simulink model "turbo_controller"  (R2025a)
settings: Solver=FixedStepAuto  StartTime=0.0  StopTime=inf  FixedStep=0.001  RelTol=1e-3
PostLoadFcn:
  | % 自动定位同目录CubeMX文件；不需要外部初始化脚本。
  | codertarget.data.setParameterValue('turbo_controller','STM32CubeMX.ProjectFile',fullfile(fileparts(get_param('turbo_controller','FileName')),'turbo_f407.ioc'));
InitFcn:
  | % 中文说明：按原控制器字段与类型创建三组接口总线；控制参数已内嵌。
  | tc_names=["EValve_Cycle" "EValve_Open" "Eblast_Cycle" "Eblast_Open" "Motor_Cycle" "Motor_Open" "EValve_Enable" "Eblast_Enable" "Motor_Enable" "SWO_Firework" "SWO_BleedAir" "EngineState" "Flag_ECUReset_Clear" "Flag_ECUReset_Save" "Flag_Reset_Enable" "Accelerator" "Nc_dem" "Nc"]; tc_types=["uint16" "uint16" "uint16" "uint16" "uint16" "uint16" "uint8" "uint8" "uint8" "uint8" "uint8" "uint8" "uint8" "uint8" "uint8" "single" "single" "single"];
  | for tc_k=1:numel(tc_names)
  |  tc_e(tc_k)=Simulink.BusElement; tc_e(tc_k).Name=char(tc_names(tc_k)); tc_e(tc_k).DataType=char(tc_types(tc_k));
  | end
  | EngineControl_Out=Simulink.Bus; EngineControl_Out.DataScope='Exported'; EngineControl_Out.Elements=tc_e;
  | clear tc_e tc_names tc_types tc_k
  | tc_names=["savedata1" "savedata2" "savedata3" "savedata4" "savedata5" "savedata6" "savedata7" "savedata8" "savedata9" "savedata10" "savedata11" "savedata12" "savedata13" "savedata14" "savedata15" "savedata16" "savedata17" "savedata18" "savedata19" "savedata20" "savedata21" "savedata22" "savedata23" "savedata24" "savedata25"]; tc_types=["single" "single" "single" "single" "single" "single" "single" "single" "single" "single" "single" "single" "single" "single" "single" "single" "single" "single" "single" "single" "single" "single" "single" "single" "single"];
  | for tc_k=1:numel(tc_names)
  |  tc_e(tc_k)=Simulink.BusElement; tc_e(tc_k).Name=char(tc_names(tc_k)); tc_e(tc_k).DataType=char(tc_types(tc_k));
  | end
  | SaveData_Out=Simulink.Bus; SaveData_Out.DataScope='Exported'; SaveData_Out.Elements=tc_e;
  | clear tc_e tc_names tc_types tc_k
  | tc_names=["senddata1" "senddata2" "senddata3" "senddata4" "senddata5" "senddata6" "senddata7" "senddata8" "senddata9" "senddata10" "senddata11" "senddata12" "senddata13" "senddata14" "senddata15" "senddata16" "senddata17" "senddata18" "senddata19" "senddata20" "senddata21" "senddata22" "senddata23" "senddata24" "senddata25" "senddata26" "senddata27" "senddata28" "senddata29"]; tc_types=["uint8" "uint8" "uint8" "uint8" "uint8" "uint8" "uint8" "uint8" "uint8" "uint8" "uint8" "uint8" "uint8" "uint8" "uint8" "uint8" "uint8" "uint8" "uint8" "uint8" "uint8" "uint8" "uint8" "uint8" "uint8" "uint8" "uint8" "uint8" "uint8"];
  | for tc_k=1:numel(tc_names)
  |  tc_e(tc_k)=Simulink.BusElement; tc_e(tc_k).Name=char(tc_names(tc_k)); tc_e(tc_k).DataType=char(tc_types(tc_k));
  | end
  | SendData_Out=Simulink.Bus; SendData_Out.DataScope='Exported'; SendData_Out.Elements=tc_e;
  | clear tc_e tc_names tc_types tc_k
  | 
  | % 以下为接口中文说明；只设置描述，不改变数值或数据类型。
  | EngineControl_Out.Description='执行控制输出（阀、电机、点火、状态及复位请求）';
  | tc_cn=["EValve_Cycle（主油阀周期计数（每计数2毫秒））" "EValve_Open（主油阀开通计数（每计数2毫秒））" "Eblast_Cycle（副油阀周期计数（每计数2毫秒））" "Eblast_Open（副油阀开通计数（每计数2毫秒））" "Motor_Cycle（起动电机周期计数）" "Motor_Open（起动电机开通计数）" "EValve_Enable（主油阀驱动使能）" "Eblast_Enable（副油阀驱动使能）" "Motor_Enable（起动电机使能）" "SWO_Firework（点火器使能（1开））" "SWO_BleedAir（引气阀使能（1开））" "EngineState（发动机状态）" "Flag_ECUReset_Clear（清除复位恢复状态请求）" "Flag_ECUReset_Save（保存复位恢复数据请求）" "Flag_Reset_Enable（处理器软件复位请求）" "Accelerator（油门／油泵给定控制量）" "Nc_dem（控制目标转速）" "Nc（发动机反馈转速（转每分））"];
  | tc_elements=EngineControl_Out.Elements;
  | for tc_k=1:numel(tc_cn)
  |  tc_elements(tc_k).Description=char(tc_cn(tc_k));
  | end
  | EngineControl_Out.Elements=tc_elements;
  | clear tc_cn tc_elements tc_k
  | SaveData_Out.Description='25项运行记录；字段含义按当前模型数据来源解释';
  | tc_cn=["savedata1（指令回显记录）" "savedata2（入口总温记录（℃））" "savedata3（电源电压记录）" "savedata4（排气温度记录（℃））" "savedata5（标定燃油压力记录）" "savedata6（副油阀占空比记录（％））" "savedata7（主油阀占空比记录（％））" "savedata8（温度修正转速记录）" "savedata9（开关输出及反馈位域）" "savedata10（物理转速记录）" "savedata11（油泵目标给定原始值）" "savedata12（起动电机占空比记录（％））" "savedata13（发动机状态码记录）" "savedata14（故障告警位域记录）" "savedata15（模型记录帧序号）" "savedata16（处理器温度记录（℃））" "savedata17（装订转速记录（沿用旧电源字段名））" "savedata18（导航高度记录）" "savedata19（飞行空速记录）" "savedata20（主阀旧记录位（恒零保留））" "savedata21（第21项保留记录（恒零））" "savedata22（保留记录项22）" "savedata23（保留记录项23）" "savedata24（保留记录项24）" "savedata25（保留记录项25）"];
  | tc_elements=SaveData_Out.Elements;
  | for tc_k=1:numel(tc_cn)
  |  tc_elements(tc_k).Description=char(tc_cn(tc_k));
  | end
  | SaveData_Out.Elements=tc_elements;
  | clear tc_cn tc_elements tc_k
  | SendData_Out.Description='29字段回传及外设命令接口；板端上位机帧只取第3至27字段';
  | tc_cn=["senddata1（回传发送允许标志（不直接上线路））" "senddata2（回传载荷长度25字节）" "senddata3（回传指令回显字节）" "senddata4（总温编码字节（℃＋80））" "senddata5（电源电压编码字节）" "senddata6（排温编码高字节）" "senddata7（排温编码低字节）" "senddata8（燃油压力编码高字节）" "senddata9（燃油压力编码低字节）" "senddata10（副油阀占空比字节（％））" "senddata11（主油阀占空比字节（％））" "senddata12（修正转速编码高字节）" "senddata13（修正转速编码低字节）" "senddata14（驱动及反馈状态位域）" "senddata15（物理转速编码高字节）" "senddata16（物理转速编码低字节）" "senddata17（油泵目标给定高字节（串口二使用））" "senddata18（油泵目标给定低字节（串口二使用））" "senddata19（起动电机占空比命令（串口一使用））" "senddata20（发动机状态码字节）" "senddata21（故障告警位域字节）" "senddata22（帧序号占位（板端另行填写））" "senddata23（处理器温度编码（℃＋50））" "senddata24（控制目标转速编码高字节）" "senddata25（控制目标转速编码低字节）" "senddata26（占位字节（板端改填实测泵速高字节））" "senddata27（占位字节（板端改填实测泵速低字节））" "senddata28（装订转速高字节（本板未发送））" "senddata29（装订转速低字节（本板未发送））"];
  | tc_elements=SendData_Out.Elements;
  | for tc_k=1:numel(tc_cn)
  |  tc_elements(tc_k).Description=char(tc_cn(tc_k));
  | end
  | SendData_Out.Elements=tc_elements;
  | clear tc_cn tc_elements tc_k
  | 
  | 
  | % FRAM模块化事务：接口类型和上电初始状态，随模型保存，无外部初始化文件。
  | clear FM_elements
  | FM_elements(1)=Simulink.BusElement;FM_elements(1).Name='phase';FM_elements(1).DataType='uint8';FM_elements(1).Dimensions=[1 1];FM_elements(1).Description='phase（当前事务阶段）';
  | FM_elements(2)=Simulink.BusElement;FM_elements(2).Name='a';FM_elements(2).DataType='uint8';FM_elements(2).Dimensions=[64 1];FM_elements(2).Description='a（启动时缓存的首区64字节）';
  | FM_elements(3)=Simulink.BusElement;FM_elements(3).Name='active';FM_elements(3).DataType='uint16';FM_elements(3).Dimensions=[1 1];FM_elements(3).Description='active（当前有效记录区地址）';
  | FM_elements(4)=Simulink.BusElement;FM_elements(4).Name='generation';FM_elements(4).DataType='uint32';FM_elements(4).Dimensions=[1 1];FM_elements(4).Description='generation（当前有效记录代号）';
  | FM_elements(5)=Simulink.BusElement;FM_elements(5).Name='record';FM_elements(5).DataType='uint8';FM_elements(5).Dimensions=[64 1];FM_elements(5).Description='record（本次冻结的待写记录）';
  | FM_elements(6)=Simulink.BusElement;FM_elements(6).Name='addr';FM_elements(6).DataType='uint16';FM_elements(6).Dimensions=[1 1];FM_elements(6).Description='addr（本次备用写入地址）';
  | FM_elements(7)=Simulink.BusElement;FM_elements(7).Name='lastSave';FM_elements(7).DataType='single';FM_elements(7).Dimensions=[1 1];FM_elements(7).Description='lastSave（上次开始保存的秒数）';
  | FM_elements(8)=Simulink.BusElement;FM_elements(8).Name='lastState';FM_elements(8).DataType='uint8';FM_elements(8).Dimensions=[1 1];FM_elements(8).Description='lastState（上次保存时的发动机状态）';
  | FM_elements(9)=Simulink.BusElement;FM_elements(9).Name='boot';FM_elements(9).DataType='boolean';FM_elements(9).Dimensions=[1 1];FM_elements(9).Description='boot（启动记录是否允许恢复）';
  | FM_elements(10)=Simulink.BusElement;FM_elements(10).Name='consumed';FM_elements(10).DataType='boolean';FM_elements(10).Dimensions=[1 1];FM_elements(10).Description='consumed（本次启动恢复通知是否已发送）';
  | FM_elements(11)=Simulink.BusElement;FM_elements(11).Name='payload';FM_elements(11).DataType='uint8';FM_elements(11).Dimensions=[20 1];FM_elements(11).Description='payload（当前20字节恢复内容）';
  | ... (+35 lines)
model workspace (MAT data in the model file):
  CRC16_Table_Reference = [0 4129 8258 12387 16516 20645 24774 28903 33032 37161 41290 45419 ... (256 elements, 256x1)]
  PE_Kaer = [0.15402 0.15402 0.12264 0.10076 0.09481 0.07601 0.07111 0.0569 0.05198 0.04926 0.05308 0.04325 ... (13 elements, 1x13)]
  PE_Nr = [21.2982 61.4260372 67.7475458 72.7394382 76.845934 80.6988798 83.8449282 86.6491912 88.9382406 89.178606 91.1938214 93.4068058 ... (13 elements, 1x13)]
  PE_Pump_Translate = 33.5999984741
  PE_RotaSpeed_Translate = 860
  PE_Taer = [0.4939154 0.4939154 0.40780982 0.34066978 0.31622756 0.30405716 0.34300244 0.26785022 0.37393554 0.23914836 0.44563948 0.31044662 ... (13 elements, 1x13)]
  PF_ACCFULLRANGE = 3360
  PF_Flag_ECUReset = 0
  PF_Flag_rx_suc = 1
  PF_Gear_Info = [40000; 45000; 50000; 55000; 57000; 59000; 60000; 61000; 61000; 61000; 61000; 61000]
  PF_K_TiaoJie = 1
  PF_Kpu = 10
  PF_MySet_Rxdata = [0 0 0 0 0 0 0 0 0 0 0 0 ... (50 elements, 50x1)]
  PF_MyUsart1_Rxdata = [0 0 0 0 0 0 0 0 0 0 0 0 ... (50 elements, 50x1)]
  PF_MyUsart2_Rxdata = [0 0 0 0 0 0 0 0 0 0 0 0 ... (50 elements, 50x1)]
  PF_Reset_Information = [0 0 0 0 0 0 0 0 0 0 0 0 ... (20 elements, 20x1)]
  PF_Sensor_X1_T4 = [0 4095]
  PF_Sensor_X2_T4 = [0 1.66666698456]
  PF_Sensor_X3_T4 = [0 504 999 1497 2010 2529 3051 3568 4076 4571 4959]
  PF_Sensor_X_P2 = [0.5 3]
  PF_Sensor_X_Poil = [0.5 3]
  PF_Sensor_X_T1t = [-50 300]
  PF_Sensor_X_Vpower = [0 3]
  PF_Sensor_X_Vpump = [0 3]
  PF_Sensor_Y1_T4 = [0 3]
  PF_Sensor_Y2_T4 = [0 5000]
  PF_Sensor_Y3_T4 = [0 100 200 300 400 500 600 700 800 900 980]
  PF_Sensor_Y_P2 = [0 1000]
  PF_Sensor_Y_Poil = [0 1000]
  PF_Sensor_Y_T1t = [-50 300]
  PF_Sensor_Y_Vpower = [0 33]
  PF_Sensor_Y_Vpump = [0 33]
  PG_CtrlMode_CloseLoop : mpt.Parameter (value not decoded)
  PG_CtrlMode_ManualAcc : mpt.Parameter (value not decoded)
  PG_CtrlMode_Origin : mpt.Parameter (value not decoded)
  PG_CtrlMode_Start : mpt.Parameter (value not decoded)
  PG_CtrlMode_Stop : mpt.Parameter (value not decoded)
  PG_ES_Clp : mpt.Parameter (value not decoded)
  PG_ES_EngStart : mpt.Parameter (value not decoded)
  PG_ES_Manual : mpt.Parameter (value not decoded)
  PG_ES_Origin : mpt.Parameter (value not decoded)
  PG_ES_Stop : mpt.Parameter (value not decoded)
  PG_Instr_BleedAirSet : mpt.Parameter (value not decoded)
  PG_Instr_CloseLoop : mpt.Parameter (value not decoded)
  PG_Instr_ECUReSet : mpt.Parameter (value not decoded)
  PG_Instr_EValveSet : mpt.Parameter (value not decoded)
  PG_Instr_EblastSet : mpt.Parameter (value not decoded)
  PG_Instr_Erase : mpt.Parameter (value not decoded)
  PG_Instr_FireWorkSet : mpt.Parameter (value not decoded)
  PG_Instr_ManualPlus : mpt.Parameter (value not decoded)
  PG_Instr_ManualrReduce : mpt.Parameter (value not decoded)
  PG_Instr_MotorSet : mpt.Parameter (value not decoded)
  PG_Instr_OilSet : mpt.Parameter (value not decoded)
  PG_Instr_SelfCheck : mpt.Parameter (value not decoded)
  PG_Instr_Start : mpt.Parameter (value not decoded)
  PG_Instr_Stop : mpt.Parameter (value not decoded)
  PG_Instr_StopZero : Simulink.Parameter (value not decoded)
  PG_Location_Air : Simulink.Parameter (value not decoded)
  PG_Location_Gnd : Simulink.Parameter (value not decoded)
  PG_ServoCtrlMode_CloseLoop : Simulink.Parameter (value not decoded)
  PG_ServoCtrlMode_CloseLoopMax : Simulink.Parameter (value not decoded)
  PG_ServoCtrlMode_CloseLoopMin : Simulink.Parameter (value not decoded)
  PG_ServoCtrlMode_ManualAcc : Simulink.Parameter (value not decoded)
  PG_ServoCtrlMode_ManualAccMax : Simulink.Parameter (value not decoded)
  PG_ServoCtrlMode_ManualAccMin : Simulink.Parameter (value not decoded)
  PG_SpeedDot_Permit : Simulink.Parameter (value not decoded)
  PL_EngineModel_Actuator = [0 10 100]
  PL_EngineModel_EngineStar_Press_P2 = [1013 1098.4 1099.144828 1099.931034 1103.613793 1162.662069 1143.793103 1131.006897 1123.186207 1117.6 1114 1111.806897 ... (127 elements, 1x127)]
  PL_EngineModel_EngineStar_RotaSpeed = [200 2000 9584 9660 10220 10240 10260 10288 10308 10368 10380 10408 ... (127 elements, 1x127)]
  PL_EngineModel_EngineStar_Temp_Exhaust = [128 129 129.1 130 131 131.1 132 133 134 134.1 135 135.1 ... (127 elements, 1x127)]
  PL_EngineModel_EngineStar_Time = [0.05 0.1 0.15 0.2 0.25 0.3 0.35 0.4 0.45 0.5 0.55 0.6 ... (127 elements, 1x127)]
  PL_EngineModel_IdleAbove_Nr = [0 21.2982 61.4260372 67.7475458 72.7394382 76.845934 80.6988798 83.8449282 86.6491912 88.9382406 89.178606 91.1938214 ... (14 elements, 1x14)]
  PL_EngineModel_IdleAbove_P2r = [0.986923266716 1.57907722675 1.81593881076 1.99358499877 2.23044658278 2.43770046879 2.65482358747 2.84233900814 3.03972366149 3.18776215149 3.25684678016 3.3950160375 ... (14 elements, 1x14)]
  PL_EngineModel_IdleAbove_Tempr = [0.0536001429337 1.07200285867 1.63301768805 1.63659103091 1.66875111667 1.72592460247 1.77595140254 1.86171163123 1.95461854565 2.03323208862 2.03323208862 2.13685903162 ... (14 elements, 1x14)]
  PL_EngineModel_IdleAbove_Ter = [0.42434128 0.42434128 0.42434128 0.30669408 0.23570008 0.22150128 0.1997974 0.23803274 0.16115638 0.24279948 0.13600422 0.31308354 ... (14 elements, 1x14)]
  PL_EngineModel_IdleAbove_Wfr = [0 10.142 23.8337 27.8905 31.9473 36.0041 40.0609 44.1177 48.1745 52.2313 52.7384 56.7952 ... (14 elements, 1x14)]
  PL_EngineModel_Press_P2 = [400 400 400 400 400 400 400 400 400 400]
  PL_EngineModel_Rotaspeed = [0 20000 96400]
  PL_EngineModel_Temp_Exhaust = [500 500 500 500 500 500 500 500 500 500]
  PL_Kaer = [0.1 0.1 0.1 0.1 0.1 0.1]
  PL_Nr = [50 60 70 80 90 100]
  PL_Taer = [0.1 0.1 0.1 0.1 0.1 0.1]
  Sig : Simulink.Signal (value not decoded)
  Ts_ms : Simulink.Parameter (value not decoded)
  false : Simulink.Parameter (value not decoded)
  true : Simulink.Parameter (value not decoded)
symbols that are objects in the model workspace (value not decoded): PG_CtrlMode_CloseLoop, PG_CtrlMode_ManualAcc, PG_CtrlMode_Origin, PG_CtrlMode_Start, PG_CtrlMode_Stop, PG_ES_Clp, PG_ES_EngStart, PG_ES_Manual, PG_ES_Origin, PG_ES_Stop, PG_Instr_BleedAirSet, PG_Instr_CloseLoop, PG_Instr_EblastSet, PG_Instr_ECUReSet, PG_Instr_Erase, PG_Instr_EValveSet, PG_Instr_FireWorkSet, PG_Instr_ManualPlus, PG_Instr_ManualrReduce, PG_Instr_MotorSet, PG_Instr_OilSet, PG_Instr_SelfCheck, PG_Instr_Start, PG_Instr_Stop, PG_Instr_StopZero, PG_ServoCtrlMode_CloseLoop, PG_ServoCtrlMode_CloseLoopMax, PG_ServoCtrlMode_CloseLoopMin, PG_ServoCtrlMode_ManualAcc, PG_ServoCtrlMode_ManualAccMax, PG_ServoCtrlMode_ManualAccMin, Ts_ms
libraries: simulink x97, stm32blockslib x10, stm32f4xxblockslib x8
(part 20 of 26)

== system turbo_controller/CLM/Start/Subsystem/If Action Subsystem ==
  note: 在参数切换前继续使用上一组起动曲线
      |
      | 本分支把输入的m1、m2、m3、m4、n1、n2按原顺序打成参数总线，不改变其数值。上层条件选择本分支
      | 时，普通起动继续沿用此前保存的曲线。
      |
      | 例如旧m1为1600，本分支仍输出1600，不会根据当前压力重新计算。压力查表更新在另一个动作分支完
      | 成；两条分支由父级If选择后汇合，不能把两组参数相加。
  In1 : Inport
      settings: AttributesFormatString=In1（输入1）
  In2 : Inport  Port=2
      settings: AttributesFormatString=In2（输入2）
  In3 : Inport  Port=3
      settings: AttributesFormatString=In3（输入3）
  In4 : Inport  Port=4
      settings: AttributesFormatString=In4（输入4）
  In5 : Inport  Port=5
      settings: AttributesFormatString=In5（输入5）
  In6 : Inport  Port=6
      settings: AttributesFormatString=In6（输入6）
  Action Port : ActionPort  ActionPortLabel=if(u1 > 0)
      settings: AttributesFormatString=Action Port（动作端口）
  Out1 : Outport
      settings: AttributesFormatString=Out1（输出1）
  Out2 : Outport  Port=2
      settings: AttributesFormatString=Out2（输出2）
  Out3 : Outport  Port=3
      settings: AttributesFormatString=Out3（输出3）
  Out4 : Outport  Port=4
      settings: AttributesFormatString=Out4（输出4）
  Out5 : Outport  Port=5
      settings: AttributesFormatString=Out5（输出5）
  Out6 : Outport  Port=6
      settings: AttributesFormatString=Out6（输出6）
  wires:
  In1/1 -> Out1/1
  In4/1 -> Out4/1
  In2/1 -> Out2/1
  In3/1 -> Out3/1
  In6/1 -> Out6/1
  In5/1 -> Out5/1

== system turbo_controller/CLM/Start/Subsystem/If Action Subsystem1 ==
  note: 根据滤波燃油压力生成普通起动的供油曲线
      |
      | 使用滤波燃油压力50和100两个断点线性插值。对应参数分别为：
      | m1：1600→1900；m2：1700→2500；
      | m3：1900→2700；m4：1500→2300；
      | n1：8800→7000；n2固定20000 rpm。
      |
      | 例如压力处于两个断点正中间75时，m1=1750、m2=2100、m3=2300、m4=1900、n1=7900。m是泵控制编码
      | ，n是阶段转速参数。生成的六项打成一组送起动顺序图，后者再结合当前转速计算实际给定。
  P : Inport
      settings: AttributesFormatString=P（压力或比例变量）
  Action Port : ActionPort  ActionPortLabel=else
      settings: AttributesFormatString=Action Port（动作端口）
  Constant : Constant  Value=[1600 1900]  OutDataTypeStr=single
      settings: AttributesFormatString=Constant（常量）
  Constant{1,3,5,7,9} (5 alike) : Constant  Value=[50 100]  OutDataTypeStr=single
      Constant1 settings: AttributesFormatString=Constant1（常量1）
      Constant3 settings: AttributesFormatString=Constant3（常量3）
      Constant5 settings: AttributesFormatString=Constant5（常量5）
      Constant7 settings: AttributesFormatString=Constant7（常量7）
      Constant9 settings: AttributesFormatString=Constant9（常量9）
  Constant10 : Constant  Value=20000  OutDataTypeStr=single
      settings: AttributesFormatString=Constant10（常量10）
  Constant2 : Constant  Value=[1700 2500]  OutDataTypeStr=single
      settings: AttributesFormatString=Constant2（常量2）
  Constant4 : Constant  Value=[1900 2700]  OutDataTypeStr=single
      settings: AttributesFormatString=Constant4（常量4）
  Constant6 : Constant  Value=[1500 2300]  OutDataTypeStr=single
      settings: AttributesFormatString=Constant6（常量6）
  Constant8 : Constant  Value=[8800 7000]  OutDataTypeStr=single
      settings: AttributesFormatString=Constant8（常量8）
  Lookup Table Dynamic{,1..4} (5 alike) : simulink/Lookup Tables/Lookup Table Dynamic  LookUpMeth=Interpolation-Use End Values  OutDataType=fixdt('single')  OutScaling=[]  OutputDataTypeScalingMode=Specify via dialog  OutDataTypeStr=fixdt('single')  DoSatur=off
      Lookup Table Dynamic settings: AttributesFormatString=Lookup Table Dynamic（动态查表）
      Lookup Table Dynamic1 settings: AttributesFormatString=Lookup Table Dynamic1（动态查表1）
      Lookup Table Dynamic2 settings: AttributesFormatString=Lookup Table Dynamic2（动态查表2）
      Lookup Table Dynamic3 settings: AttributesFormatString=Lookup Table Dynamic3（动态查表3）
      Lookup Table Dynamic4 settings: AttributesFormatString=Lookup Table Dynamic4（动态查表4）
  Scope : Scope
      settings: AttributesFormatString=Scope（示波器）  ActiveDisplayYMinimum=1892.31507  ActiveDisplayYMaximum=1910.29465  DataLoggingVariableName=ScopeData2
  m1 : Outport
      settings: AttributesFormatString=m1（中位或中间变量1）
  m2 : Outport  Port=2
      settings: AttributesFormatString=m2（中位或中间变量2）
  m3 : Outport  Port=3
      settings: AttributesFormatString=m3（中位或中间变量3）
  m4 : Outport  Port=4
      settings: AttributesFormatString=m4（中位或中间变量4）
  n1 : Outport  Port=5
      settings: AttributesFormatString=n1（转速变量1）
  n2 : Outport  Port=6
      settings: AttributesFormatString=n2（转速变量2）
  wires:
  Constant1/1 -> Lookup Table Dynamic/2
  Constant/1 -> Lookup Table Dynamic/3
  P/1 -> Lookup Table Dynamic4/1, Lookup Table Dynamic3/1, Lookup Table Dynamic2/1, Lookup Table Dynamic1/1, Lookup Table Dynamic/1
  Constant2/1 -> Lookup Table Dynamic1/3
  Constant4/1 -> Lookup Table Dynamic2/3
  Constant6/1 -> Lookup Table Dynamic3/3
  Constant3/1 -> Lookup Table Dynamic1/2
  Constant5/1 -> Lookup Table Dynamic2/2
  Constant7/1 -> Lookup Table Dynamic3/2
  Lookup Table Dynamic/1 -> m1/1, Scope/1
  Lookup Table Dynamic1/1 -> m2/1
  Lookup Table Dynamic2/1 -> m3/1
  Lookup Table Dynamic3/1 -> m4/1
  Constant8/1 -> Lookup Table Dynamic4/3
  Constant9/1 -> Lookup Table Dynamic4/2
  Lookup Table Dynamic4/1 -> n1/1
  Constant10/1 -> n2/1

== system turbo_controller/COMMRead_ISM/CMMRead/Instr_Analyse/装订和档位控制 ==
  note: 【本页库子系统中文说明】dangwei
      | 一、它做什么？
      | 这是“过不过这条线”的判断器。将输入与阈值 uint8(hex2dec('0D')) 作 == 比较，
      | 关系成立输出真（1），否则输出假（0）。例如>=包含恰好等于，>则不包含。它只给
      | 出判断标志，不会自行限幅、报警、切换状态或操作阀门；后续逻辑决定如何使用。名
      | 称可能只是用途提示，实际判据以这里的关系和阈值为准。
      | 二、本实例当前参数
      | 比较关系：==
      | 比较阈值：uint8(hex2dec('0D'))
      | 输出数据类型：uint8
      | 零交叉检测：开启
      | 三、怎样继续学习？
      | 这是标准库子系统实例。中文说明放在使用它的父级页面，并同步存入本块Descriptio
      | n（模块说明）；官方库链接保留。先看本实例的输入来自哪里、输出交给谁，再结合
      | 以上参数理解作用。
  note: 【本页库子系统中文说明】zhuangding
      | 一、它做什么？
      | 这是“过不过这条线”的判断器。将输入与阈值 uint8(hex2dec('F3')) 作 == 比较，
      | 关系成立输出真（1），否则输出假（0）。例如>=包含恰好等于，>则不包含。它只给
      | 出判断标志，不会自行限幅、报警、切换状态或操作阀门；后续逻辑决定如何使用。名
      | 称可能只是用途提示，实际判据以这里的关系和阈值为准。
      | 二、本实例当前参数
      | 比较关系：==
      | 比较阈值：uint8(hex2dec('F3'))
      | 输出数据类型：uint8
      | 零交叉检测：开启
      | 三、怎样继续学习？
      | 这是标准库子系统实例。中文说明放在使用它的父级页面，并同步存入本块Descriptio
      | n（模块说明）；官方库链接保留。先看本实例的输入来自哪里、输出交给谁，再结合
      | 以上参数理解作用。
  note: 【本页库子系统中文说明】取高8位
      | 一、它做什么？
      | 从一个整数里取出部分二进制位，相当于把一串数字中的固定位置剪出来。当前取位范
      | 围为 [0 7]，位编号从0开始。范围[0 7]是低字节，[8 15]是高字节；取出的位按整数
      | 解释，便于组通信帧或运行记录。它不是额外测量一次，也不是计算平均值。
      | 二、本实例当前参数
      | 取位方式：Upper half
      | 位数：8
      | 位编号范围：[0 7]
      | 取出的位如何解释：把选出的位当成一个整数
      | 三、怎样继续学习？
      | 这是标准库子系统实例。中文说明放在使用它的父级页面，并同步存入本块Descriptio
      | n（模块说明）；官方库链接保留。先看本实例的输入来自哪里、输出交给谁，再结合
      | 以上参数理解作用。
  note: 【本页库子系统中文说明】最大档位
      | 一、它做什么？
      | 这是“过不过这条线”的判断器。将输入与阈值 uint8(12) 作 <= 比较，关系成立输
      | 出真（1），否则输出假（0）。例如>=包含恰好等于，>则不包含。它只给出判断标志
      | ，不会自行限幅、报警、切换状态或操作阀门；后续逻辑决定如何使用。名称可能只是
      | 用途提示，实际判据以这里的关系和阈值为准。
      | 二、本实例当前参数
      | 比较关系：<=
      | 比较阈值：uint8(12)
      | 输出数据类型：uint8
      | 零交叉检测：开启
      | 三、怎样继续学习？
      | 这是标准库子系统实例。中文说明放在使用它的父级页面，并同步存入本块Descriptio
      | n（模块说明）；官方库链接保留。先看本实例的输入来自哪里、输出交给谁，再结合
      | 以上参数理解作用。
  note: 判断这帧是否在设置目标转速或选择档位
      |
      | 两类编码被视为装订/档位指令：一类是命令值F3（十六进制）的直接装订；另一类是低8位为0D且取出
      | 的高8位档位号不超过12的档位命令。
      |
      | 这里仅输出“属于这一类命令”的布尔标志，不计算具体转速。具体目标由Speed_Load_Cal继续从第5
      | 、6字节或档位表取出。例：直接装订F3可以进入目标解析，普通阀门命令不会因携带了数值就变成闭
      | 环目标。
  note: dangwei
      | dangwei：只判断一个条件
      |
      | 把输入与0x0D（十进制13）比较，使用关系“==”。成立输出1，不成立输出0；输出是判断标志，不是
      | 把输入缩放成该常数。
      |
      | 这里识别一种指令编码。判断成立只说明指令匹配；父级还会结合有效帧、当前模式或其他允许条件决
      | 定是否更新。实际驱动要继续经过控制与板级输出，不能把1理解为硬件执行回执。
  note: zhuangding
      | zhuangding：只判断一个条件
      |
      | 把输入与0xF3（十进制243）比较，使用关系“==”。成立输出1，不成立输出0；输出是判断标志，不
      | 是把输入缩放成该常数。
      |
      | 这里识别一种指令编码。判断成立只说明指令匹配；父级还会结合有效帧、当前模式或其他允许条件决
      | 定是否更新。实际驱动要继续经过控制与板级输出，不能把1理解为硬件执行回执。
  note: 取高8位
      | 取高8位：从整数编码中取出指定二进制位
      |
      | 当前选择Upper half，位范围[0 7]，输出按整数解释。位号从0开始，0是最低位。它不是按十进制字
      | 符截取，也不改变传感器标定。
      |
      | 取低8位：结果=原整数 mod 256。例如1000（十六进制03E8）取出232。
      |
      | 用于回传拆字节时，高低字节要按协议顺序发送；接收方按“高×256+低”才能还原原整数。
  note: 最大档位
      | 最大档位：只判断一个条件
      |
      | 把输入与uint8(12)比较，使用关系“<=”。成立输出1，不成立输出0；输出是判断标志，不是把输入
      | 缩放成该常数。
      |
      | 比较门限用于父级的分支条件，没有滤波、延时确认或锁存。例如输入恰好等于门限时，“>=、<=、==
      | ”成立，“>、<”不成立。是否需要持续确认或同时满足其他条件，由父级连线决定。
  S_COMM_Instr : Inport
      settings: AttributesFormatString=S_COMM_Instr（通信指令）
  dangwei : simulink/Logic and Bit Operations/Compare To Constant  Description=|  relop===  const=uint8(hex2dec('0D'))  OutDataTypeStr=uint8
      | dangwei：只判断一个条件
      | 
      | 把输入与0x0D（十进制13）比较，使用关系“==”。成立输出1，不成立输出0；输出是判断标志，不是把输入缩放成该常数。
      | 
      | 这里识别一种指令编码。判断成立只说明指令匹配；父级还会结合有效帧、当前模式或其他允许条件决定是否更新。实际驱动要继续经过控制与板级输出，不能把1理解为硬件执行回执。
      settings: AttributesFormatString=dangwei（档位）
  zhuangding : simulink/Logic and Bit Operations/Compare To Constant  Description=|  relop===  const=uint8(hex2dec('F3'))  OutDataTypeStr=uint8
      | zhuangding：只判断一个条件
      | 
      | 把输入与0xF3（十进制243）比较，使用关系“==”。成立输出1，不成立输出0；输出是判断标志，不是把输入缩放成该常数。
      | 
      | 这里识别一种指令编码。判断成立只说明指令匹配；父级还会结合有效帧、当前模式或其他允许条件决定是否更新。实际驱动要继续经过控制与板级输出，不能把1理解为硬件执行回执。
      settings: AttributesFormatString=zhuangding（装订参数）
  "低8位 " : simulink/Logic and Bit Operations/Bitwise Operator  logicop=AND  UseBitMask=on  BitMask=bin2dec('1111')  BitMaskRealWorld=Stored Integer
  取高8位 : simulink/Logic and Bit Operations/Extract Bits  Description=|  bitsToExtract=Upper half  numBits=8  bitIdxRange=[0 7]  outScalingMode=Treat bit field as an integer
      | 取高8位：从整数编码中取出指定二进制位
      | 
      | 当前选择Upper half，位范围[0 7]，输出按整数解释。位号从0开始，0是最低位。它不是按十进制字符截取，也不改变传感器标定。
      | 
      | 取低8位：结果=原整数 mod 256。例如1000（十六进制03E8）取出232。
      | 
      | 用于回传拆字节时，高低字节要按协议顺序发送；接收方按“高×256+低”才能还原原整数。
  最大档位 : simulink/Logic and Bit Operations/Compare To Constant  Description=|  relop=<=  const=uint8(12)  OutDataTypeStr=uint8
      | 最大档位：只判断一个条件
      | 
      | 把输入与uint8(12)比较，使用关系“<=”。成立输出1，不成立输出0；输出是判断标志，不是把输入缩放成该常数。
      | 
      | 比较门限用于父级的分支条件，没有滤波、延时确认或锁存。例如输入恰好等于门限时，“>=、<=、==”成立，“>、<”不成立。是否需要持续确认或同时满足其他条件，由父级连线决定。
  "档位+装订 " : Logic  Operator=OR  AllPortsSameDT=off  OutDataTypeStr=boolean
  档位范围 : Logic  AllPortsSameDT=off  OutDataTypeStr=boolean
  S_Flagf_CLP : Outport
      settings: AttributesFormatString=S_Flagf_CLP（标志闭环）
  wires:
  zhuangding/1 -> "档位+装订 "/1
  "档位+装订 "/1 -> S_Flagf_CLP/1
  "低8位 "/1 -> dangwei/1
  S_COMM_Instr/1 -> 取高8位/1, "低8位 "/1, zhuangding/1
  取高8位/1 -> 最大档位/1
  dangwei/1 -> 档位范围/1
  最大档位/1 -> 档位范围/2
  档位范围/1 -> "档位+装订 "/2

== system turbo_controller/COMMRead_ISM/CMMRead/SpeedLoad_Analyse/Speed_Load_Cal ==
  note: 【本页库子系统中文说明】dangwei
      | 一、它做什么？
      | 这是“过不过这条线”的判断器。将输入与阈值 uint8(hex2dec('0D')) 作 >= 比较，
      | 关系成立输出真（1），否则输出假（0）。例如>=包含恰好等于，>则不包含。它只给
      | 出判断标志，不会自行限幅、报警、切换状态或操作阀门；后续逻辑决定如何使用。名
      | 称可能只是用途提示，实际判据以这里的关系和阈值为准。
      | 二、本实例当前参数
      | 比较关系：>=
      | 比较阈值：uint8(hex2dec('0D'))
      | 输出数据类型：uint8
      | 零交叉检测：开启
      | 三、怎样继续学习？
      | 这是标准库子系统实例。中文说明放在使用它的父级页面，并同步存入本块Descriptio
      | n（模块说明）；官方库链接保留。先看本实例的输入来自哪里、输出交给谁，再结合
      | 以上参数理解作用。
  note: 【本页库子系统中文说明】zhuangding
      | 一、它做什么？
      | 这是“过不过这条线”的判断器。将输入与阈值 uint8(hex2dec('F3')) 作 == 比较，
      | 关系成立输出真（1），否则输出假（0）。例如>=包含恰好等于，>则不包含。它只给
      | 出判断标志，不会自行限幅、报警、切换状态或操作阀门；后续逻辑决定如何使用。名
      | 称可能只是用途提示，实际判据以这里的关系和阈值为准。
      | 二、本实例当前参数
      | 比较关系：==
      | 比较阈值：uint8(hex2dec('F3'))
      | 输出数据类型：uint8
      | 零交叉检测：开启
      | 三、怎样继续学习？
      | 这是标准库子系统实例。中文说明放在使用它的父级页面，并同步存入本块Descriptio
      | n（模块说明）；官方库链接保留。先看本实例的输入来自哪里、输出交给谁，再结合
      | 以上参数理解作用。
  note: 【本页库子系统中文说明】取高4位
      | 一、它做什么？
      | 从一个整数里取出部分二进制位，相当于把一串数字中的固定位置剪出来。当前取位范
      | 围为 [0 7]，位编号从0开始。范围[0 7]是低字节，[8 15]是高字节；取出的位按整数
      | 解释，便于组通信帧或运行记录。它不是额外测量一次，也不是计算平均值。
      | 二、本实例当前参数
      | 取位方式：Upper half
      | 位数：8
      | 位编号范围：[0 7]
      | 取出的位如何解释：把选出的位当成一个整数
      | 三、怎样继续学习？
      | 这是标准库子系统实例。中文说明放在使用它的父级页面，并同步存入本块Descriptio
      | n（模块说明）；官方库链接保留。先看本实例的输入来自哪里、输出交给谁，再结合
      | 以上参数理解作用。
  note: 把直接装订或档位编码换算为目标转速
      |
      | 直接装订：第3字节等于F3时，取第5、6字节，按高字节在前合成整数，再乘2。
      | 目标rpm = 2×(第5字节×256+第6字节)。
      | 例如高字节97、低字节168，合成25000，得到50000 rpm。
      |
      | 档位路径：提取第3字节的高4位作为档位索引，按模型的一基索引从PF_Gear_Info表取目标；低位判定
      | 符合档位编码才采用，否则候选输出0。父级还会进行命令有效性和40000～61000范围选择。
      |
      | 本模块只解码，不做转速闭环；无效候选0也不一定立刻把最终目标清零，父级可能保持旧目标。
  note: dangwei
      | dangwei：只判断一个条件
      |
      | 把输入与0x0D（十进制13）比较，使用关系“>=”。成立输出1，不成立输出0；输出是判断标志，不是
      | 把输入缩放成该常数。
      |
      | 这里识别一种指令编码。判断成立只说明指令匹配；父级还会结合有效帧、当前模式或其他允许条件决
      | 定是否更新。实际驱动要继续经过控制与板级输出，不能把1理解为硬件执行回执。
  note: zhuangding
      | zhuangding：只判断一个条件
      |
      | 把输入与0xF3（十进制243）比较，使用关系“==”。成立输出1，不成立输出0；输出是判断标志，不
      | 是把输入缩放成该常数。
      |
      | 这里识别一种指令编码。判断成立只说明指令匹配；父级还会结合有效帧、当前模式或其他允许条件决
      | 定是否更新。实际驱动要继续经过控制与板级输出，不能把1理解为硬件执行回执。
  note: 取高4位
      | 取高4位：从整数编码中取出指定二进制位
      |
      | 当前选择Upper half，位范围[0 7]，输出按整数解释。位号从0开始，0是最低位。它不是按十进制字
      | 符截取，也不改变传感器标定。
      |
      | 取低8位：结果=原整数 mod 256。例如1000（十六进制03E8）取出232。
      |
      | 用于回传拆字节时，高低字节要按协议顺序发送；接收方按“高×256+低”才能还原原整数。
  S_MyUsart2_Rxdata : Inport
      settings: AttributesFormatString=S_MyUsart2_Rxdata（四号串口指令缓冲区（沿用旧变量名））
  Data Type Conversion : DataTypeConversion  OutDataTypeStr=uint8  SaturateOnIntegerOverflow=off  RndMeth=Floor
      settings: AttributesFormatString=Data Type Conversion（数据类型转换）
  Selector1 : Selector  IndexMode=Zero-based  InputPortWidth=2  IndexOptions=Index vector (dialog)  Indices=[0]  OutputSizes=1
      settings: AttributesFormatString=Selector1（选择器1）
  Selector2 : Selector  IndexMode=Zero-based  InputPortWidth=2  IndexOptions=Index vector (dialog)  Indices=[1]  OutputSizes=1
      settings: AttributesFormatString=Selector2（选择器2）
  Switch : Switch  Criteria=u2 ~= 0  SaturateOnIntegerOverflow=off  InputSameDT=off
      settings: AttributesFormatString=Switch（开关选择）
  Switch1 : Switch  Criteria=u2 ~= 0  SaturateOnIntegerOverflow=off  InputSameDT=off
      settings: AttributesFormatString=Switch（开关选择）
  WuMuBiao : Constant  Value=0  OutDataTypeStr=uint32
      settings: AttributesFormatString=WuMuBiao（无目标值）
  dangwei : simulink/Logic and Bit Operations/Compare To Constant  Description=|  relop=>=  const=uint8(hex2dec('0D'))  OutDataTypeStr=uint8
      | dangwei：只判断一个条件
      | 
      | 把输入与0x0D（十进制13）比较，使用关系“>=”。成立输出1，不成立输出0；输出是判断标志，不是把输入缩放成该常数。
      | 
      | 这里识别一种指令编码。判断成立只说明指令匹配；父级还会结合有效帧、当前模式或其他允许条件决定是否更新。实际驱动要继续经过控制与板级输出，不能把1理解为硬件执行回执。
      settings: AttributesFormatString=dangwei（档位）
  zhuangding : simulink/Logic and Bit Operations/Compare To Constant  Description=|  relop===  const=uint8(hex2dec('F3'))  OutDataTypeStr=uint8
      | zhuangding：只判断一个条件
      | 
      | 把输入与0xF3（十进制243）比较，使用关系“==”。成立输出1，不成立输出0；输出是判断标志，不是把输入缩放成该常数。
      | 
      | 这里识别一种指令编码。判断成立只说明指令匹配；父级还会结合有效帧、当前模式或其他允许条件决定是否更新。实际驱动要继续经过控制与板级输出，不能把1理解为硬件执行回执。
      settings: AttributesFormatString=zhuangding（装订参数）
  乘以1 : Gain  ParamDataTypeStr=uint32  OutDataTypeStr=single
  乘以2 : Gain  Gain=2  ParamDataTypeStr=uint32  OutDataTypeStr=single
  乘以256 : Gain  Gain=hex2dec('100')  ParamDataTypeStr=uint32  OutDataTypeStr=single
  "低4位 " : simulink/Logic and Bit Operations/Bitwise Operator  logicop=AND  UseBitMask=on  BitMask=bin2dec('1111')  BitMaskRealWorld=Stored Integer
  取高4位 : simulink/Logic and Bit Operations/Extract Bits  Description=|  bitsToExtract=Upper half  numBits=8  bitIdxRange=[0 7]  outScalingMode=Treat bit field as an integer
      | 取高4位：从整数编码中取出指定二进制位
      | 
      | 当前选择Upper half，位范围[0 7]，输出按整数解释。位号从0开始，0是最低位。它不是按十进制字符截取，也不改变传感器标定。
      | 
      | 取低8位：结果=原整数 mod 256。例如1000（十六进制03E8）取出232。
      | 
      | 用于回传拆字节时，高低字节要按协议顺序发送；接收方按“高×256+低”才能还原原整数。
  档位信息1为起始位 : Selector  InputPortWidth=12  IndexOptions=Index vector (port)  Indices=[4 5]  OutputSizes=1
  档位信息数组 : Constant  Value=PF_Gear_Info
  第3字节 : Selector  IndexMode=Zero-based  InputPortWidth=50  IndexOptions=Index vector (dialog)  Indices=2  OutputSizes=1
  第5和6字节 : Selector  IndexMode=Zero-based  InputPortWidth=50  IndexOptions=Index vector (dialog)  Indices=[4 5]  OutputSizes=1
  高字节前 : Sum  AccumDataTypeStr=uint32
  S_Out_SpeedLoad : Outport
      settings: AttributesFormatString=S_Out_SpeedLoad（装订转速）
  wires:
  Selector2/1 -> 乘以1/1
  乘以256/1 -> 高字节前/1
  Selector1/1 -> 乘以256/1
  高字节前/1 -> 乘以2/1
  乘以1/1 -> 高字节前/2
  第5和6字节/1 -> Selector1/1, Selector2/1
  第3字节/1 -> zhuangding/1, 取高4位/1, "低4位 "/1
  S_MyUsart2_Rxdata/1 -> 第5和6字节/1, 第3字节/1
  "低4位 "/1 -> dangwei/1
  Switch/1 -> S_Out_SpeedLoad/1
  取高4位/1 -> Data Type Conversion/1
  档位信息数组/1 -> 档位信息1为起始位/1
  Data Type Conversion/1 -> 档位信息1为起始位/2
  Switch1/1 -> Switch/3
  乘以2/1 -> Switch/1
  zhuangding/1 -> Switch/2
  WuMuBiao/1 -> Switch1/3
  档位信息1为起始位/1 -> Switch1/1
  dangwei/1 -> Switch1/2

== system turbo_controller/COMMRead_ISM/CMMRead/T1t_P1t_Cal/Dynamic_Cal ==
  note: 由高度和空速分两步估算进气总温、总压
      |
      | 第一步P1H_T1H：输入高度H（km）、参考温度T10（K）、参考压力p10，计算该高度的静温T1H和静压P1
      | H，描述未被进气道减速前的外界空气。
      |
      | 第二步dynamic：把T1H、P1H与空速AirSpeed（m/s）一起计算，得到气流理想减速到零速度时的总温T1
      | t、总压P1t。速度越高，动能转化引起的总温与总压增加越明显。
      |
      | 例如H=0、空速=0时，总温等于参考温度，总压等于参考压力。空速不为0时，不能只按高度算静压后就
      | 把它称为总压。公式及适用假设分别写在下面两个子系统内部。
  H : Inport
      settings: AttributesFormatString=H（高度）
  AirSpeed : Inport  Port=2
      settings: AttributesFormatString=AirSpeed（空速）
  T10 : Inport  Port=3
      settings: AttributesFormatString=T10（入口参考温度）
  p10 : Inport  Port=4
      settings: AttributesFormatString=p10（压力或比例变量10）
  Data Type Conversion1 : DataTypeConversion  OutDataTypeStr=single  SaturateOnIntegerOverflow=off  RndMeth=Floor
      settings: AttributesFormatString=Data Type Conversion1（数据类型转换1）
  Data Type Conversion5 : DataTypeConversion  OutDataTypeStr=single  SaturateOnIntegerOverflow=off  RndMeth=Floor
      settings: AttributesFormatString=Data Type Conversion5（数据类型转换5）
  P1H_T1H : Subsystem  Description=|
      | 按分层标准大气关系计算高度处静温和静压
      | 
      | H采用km，温度采用K。11 km以下采用每升高1 km降温6.5 K的近似：
      | T1H = T10 - 6.5×H；
      | P1H = p10×(1-0.022577×H)^5.25588。
      | 
      | 11 km及以上采用本模型的等温层近似：
      | T1H = T10 - 6.5×11；
      | P1H = 23.385×exp[-0.1576932×(H-11)]（kPa）。
      | 高空压力支路使用固定23.385 kPa，并不再乘参考压力p10。因此两层交界处按当前系数并非严格连续；这里如实说明现有计算，没有调整算法。
      | 
      | 低层公式体现温度递减条件下的静力平衡：越高，上方空气柱越少，压力降低。高层近似温度不再下降，压力按指数衰减。标准参考T10=288.15 K、p10=101.325时，海平面输出288.15 K与101.325；11 km处温度216.65 K。
      | 
      | 这是高度大气近似，不包含天气、湿度和进气损失。当前没有由此自动识别超出适用高度范围的传感器故障。
      settings: AttributesFormatString=P1H_T1H（对应高度的入口压力对应高度的入口温度）
  "dynamic " : Subsystem  Description=|
      | 把飞行空速对应的动能计入进气总温、总压
      | 
      | 输入静温T1H（K）、静压P1H和空速V=AirSpeed（m/s）。先求当地声速，再求马赫数：
      | a = sqrt(1.4×287.06×T1H)；
      | M = V/a。
      | 1.4为空气比热比，287.06是空气气体常数，a的单位m/s。M表示飞行速度是当地声速的多少倍，不是把空速直接除以固定340。
      | 
      | 再计算理想气流减速后的总量：
      | 温升因子 = 1+0.2×M²；
      | T1t = T1H×温升因子；
      | P1t = P1H×温升因子^3.5。
      | 3.5=1.4/0.4，模型恢复系数当前为1。
      | 
      | 例如静温288.15 K时声速约340.3 m/s，空速100 m/s得到M约0.294，温升因子约1.0173，总温约293.13 K；总压约为静压的1.0616倍。空速0时总温、总压回到静温、静压。
      | 
      | 公式假设理想气体和等熵减速，没有额外模拟进气道摩擦、激波或测量误差。压力单位沿用输入，不能因为计算名称含dynamic就把结果当成单独的动压。
      settings: AttributesFormatString=dynamic （动态）
  T1t : Outport
      settings: AttributesFormatString=T1t（入口总温）
  P1t : Outport  Port=2
      settings: AttributesFormatString=P1t（入口总压）
  wires:
  T10/1 -> P1H_T1H/2(T10)
  P1H_T1H/1(T1H) -> "dynamic "/1(T1H)
  P1H_T1H/2(P1H) -> "dynamic "/2(P1H)
  AirSpeed/1 -> "dynamic "/3(AirSpeed)
  "dynamic "/2(P1t) -> Data Type Conversion1/1
  "dynamic "/1(T1t) -> Data Type Conversion5/1
  p10/1 -> P1H_T1H/3(p10)
  H/1 -> P1H_T1H/1(H)
  Data Type Conversion5/1 -> T1t/1
  Data Type Conversion1/1 -> P1t/1

== system turbo_controller/COMMRead_ISM/ISM/AnalogFilter_Nc/GeneralFilter ==
  note: 先拒绝明显不可信的转速，再平滑有效值
      |
      | Xlim_Xdot_Judge比较当前原始输入、前一拍原始输入和前一拍有效输出。超出允许上下限或突变不满
      | 足接受条件时，输出沿用上次有效值，并分别标记幅值故障、变化故障。
      |
      | 恢复时不仅要求变化回到较小门限，还要达到连续确认次数。次数由恢复时间/Ts_ms计算，避免一拍恢
      | 复就马上解除故障。
      |
      | 通过检查的值再进入一阶低通，延迟同时保存本拍原始值和有效值，供下一拍比较。因此“原始上一拍
      | ”与“上一有效输出”是两条不同的记忆，不能混为一个变量。
  Xin : Inport
      settings: AttributesFormatString=Xin（输入量）
  X_ulim : Inport  Port=2
      settings: AttributesFormatString=X_ulim（输入上限）
  X_llim : Inport  Port=3
      settings: AttributesFormatString=X_llim（输入下限）
  Xdot_lim : Inport  Port=4
      settings: AttributesFormatString=Xdot_lim（变化量限值）
  Xdot_CancelLim : Inport  Port=5
      settings: AttributesFormatString=Xdot_CancelLim（输入变化量解除限值）
  Xdot_CancelTime : Inport  Port=6
      settings: AttributesFormatString=Xdot_CancelTime（输入变化量解除时间）
  Constant3 : Constant  Value=Ts_ms  OutDataTypeStr=single  SampleTime=-1
      settings: AttributesFormatString=Constant3（常量3）
  Divide1 : Product  Inputs=*/
      settings: AttributesFormatString=Divide1（除法1）
  Subsystem : Subsystem  Description=|
      | 对经过有效性判断的转速做一阶低通，减小采样抖动
      | 
      | 每次把本拍输入与上次滤波结果按比例相加：
      | 本拍输出=α×本拍输入+β×上次输出；
      | α=Ts/(T+Ts)，β=T/(T+Ts)。
      | 
      | 当前T=0.067 s，Ts=Ts_ms/1000=0.02 s，因此α约0.229885、β约0.770115。新输入约占23%，旧结果约占77%。例如上次输出100、本次输入200，本次滤波结果约123，随后逐步靠近200。
      | 
      | 它抑制快速波动，也会让真实变化稍有滞后；不负责把ADC计数变成物理量，也不单凭滤波判定传感器故障。输出送Nc_Filter，参与控制与故障处理。
  Unit Delay : UnitDelay  RequirementInfo={} %GIDa_916f694f_1fff_461f_bb2e_fdfd38f2686d  SampleTime=-1  HasFrameUpgradeWarning=on
      settings: AttributesFormatString=Unit Delay（单位延迟）
  Unit Delay1 : UnitDelay  RequirementInfo={} %GIDa_abb45954_d250_48ef_b37b_e22540a74ef8  SampleTime=-1  HasFrameUpgradeWarning=on
      settings: AttributesFormatString=Unit Delay1（单位延迟1）
  Xlim_Xdot_Judge : Stateflow chart  Description=|  RequirementInfo={} %GIDa_8241bfcd_797e_4f0b_88bb_28dc06fe45bb  TreatAsAtomicUnit=on
      | 区分转速越界与突然跳变，并控制恢复
      | 
      | 先检查当前值是否在X_llim～X_ulim内，再检查与上一拍原始值的变化。幅值超限和变化超限分别产生X_Flag_Locking与Xdot_Flag_Locking。
      | 
      | 不接受本拍样本时，输出X_pre，即上一有效输出；接受时输出当前X。这样偶发突跳不会直接冲进闭环。变化恢复采用更小的Xdot_CancelLim门限，并累计CNT_Xdot，只有超过Xdot_Cancelcycle才解除相应保持。
      | 
      | 门限由父级给定：转速变化检查使用1200，恢复门限800，确认时间100 ms换算为调用次数。比较的是相邻采样差值，不是已经除以采样周期的rpm/s，不能把1200直接标成加速度单位。
      settings: AttributesFormatString=Xlim_Xdot_Judge（输入限值输入变化量判断）
  S_X_Flag_Locking : Outport
      settings: AttributesFormatString=S_X_Flag_Locking（自变量或输入量标志锁存）
  S_Xdot_Flag_Locking : Outport  Port=2
      settings: AttributesFormatString=S_Xdot_Flag_Locking（输入变化量标志锁存）
  S_Xout : Outport  Port=3
      settings: AttributesFormatString=S_Xout（输出量）
  wires:
  Xin/1 -> Unit Delay1/1, Xlim_Xdot_Judge/1(X)
  X_ulim/1 -> Xlim_Xdot_Judge/3(X_ulim)
  X_llim/1 -> Xlim_Xdot_Judge/4(X_llim)
  Xdot_lim/1 -> Xlim_Xdot_Judge/5(Xdot_lim)
  Xdot_CancelLim/1 -> Xlim_Xdot_Judge/6(Xdot_CancelLim)
  Unit Delay1/1 -> Xlim_Xdot_Judge/2(Xin_pre)
  Xlim_Xdot_Judge/3(X_Out) -> Unit Delay/1, Subsystem/1(In1)
  Unit Delay/1 -> Xlim_Xdot_Judge/8(X_pre)
  Divide1/1 -> Xlim_Xdot_Judge/7(Xdot_Cancelcycle)
  Xdot_CancelTime/1 -> Divide1/1
  Constant3/1 -> Divide1/2
  Xlim_Xdot_Judge/1(X_Flag_Locking) -> S_X_Flag_Locking/1
  Xlim_Xdot_Judge/2(Xdot_Flag_Locking) -> S_Xdot_Flag_Locking/1
  Subsystem/1(Out1) -> S_Xout/1

== system turbo_controller/COMMRead_ISM/ISM/AnalogFilter_Poil/Subsystem1 ==
  note: 计算低通滤波中新样本的权重
      |
      | 输入T为滤波时间常数（s），T_Sampling为采样周期（s）。输出α=T_Sampling/(T+T_Sampling)，供
      | 父级乘以本拍的新输入。
      |
      | 当前T=0.067、采样周期0.02，α=0.02/0.087≈0.229885。也就是每拍只采用约23%的新值，另外约77%
      | 由历史结果补足。时间常数越大，新值权重越小，结果越平稳但响应越慢。
      |
      | 本模块只算一个无量纲系数，不含延迟，也不直接输出温度、压力或转速。两项时间输入必须使用同一
      | 单位。
  T : Inport
      settings: AttributesFormatString=T（温度、时间或真分支输入）
  T_Sampling : Inport  Port=2
      settings: AttributesFormatString=T_Sampling（采样周期）
  Constant : Constant  OutDataTypeStr=single
      settings: AttributesFormatString=Constant（常量）
  Constant2 : Constant  OutDataTypeStr=single
      settings: AttributesFormatString=Constant2（常量2）
  Divide : Product  Inputs=*/
      settings: AttributesFormatString=Divide（除法）
  Product : Product  RndMeth=Zero
      settings: AttributesFormatString=Product（乘法）
  Product1 : Product  RndMeth=Zero
      settings: AttributesFormatString=Product1（乘法1）
  Sum : Sum  Inputs=|++
      settings: AttributesFormatString=Sum（加法求和）
  Out : Outport
      settings: AttributesFormatString=Out（输出）
  wires:
  Constant/1 -> Product/1
  T_Sampling/1 -> Product/2, Sum/2
  Product/1 -> Divide/1
  Constant2/1 -> Product1/1
  T/1 -> Product1/2
  Product1/1 -> Sum/1
  Sum/1 -> Divide/2
  Divide/1 -> Out/1

== system turbo_controller/COMMRead_ISM/ISM/AnalogFilter_Poil/Subsystem2 ==
  note: 计算低通滤波中历史结果的权重
      |
      | 输入T为时间常数，T_Sampling为采样周期，两者都用s。输出β=T/(T+T_Sampling)，供父级乘以上一
      | 次滤波结果。
      |
      | 当前T=0.067、采样周期0.02，β≈0.770115；与另一支路新样本权重α≈0.229885相加为1。这样常值
      | 输入最终会稳定在原值，不会因为反复相加而不断放大。
      |
      | 本模块只计算系数，历史结果由父级延迟块保存。若把20 ms误传成20 s，权重和滤波速度都会完全改
      | 变，因此父级先将Ts_ms除以1000。
  T : Inport
      settings: AttributesFormatString=T（温度、时间或真分支输入）
  T_Sampling : Inport  Port=2
      settings: AttributesFormatString=T_Sampling（采样周期）
  Constant : Constant  OutDataTypeStr=single
      settings: AttributesFormatString=Constant（常量）
  Constant2 : Constant  OutDataTypeStr=single
      settings: AttributesFormatString=Constant2（常量2）
  Divide : Product  Inputs=*/
      settings: AttributesFormatString=Divide（除法）
  Product : Product  RndMeth=Zero
      settings: AttributesFormatString=Product（乘法）
  Product1 : Product  RndMeth=Zero
      settings: AttributesFormatString=Product1（乘法1）
  Sum : Sum  Inputs=|++
      settings: AttributesFormatString=Sum（加法求和）
  Out : Outport
      settings: AttributesFormatString=Out（输出）
  wires:
  Constant/1 -> Product/1
  T/1 -> Product/2, Product1/2
  Product/1 -> Divide/1
  Constant2/1 -> Product1/1
  Product1/1 -> Sum/1
  T_Sampling/1 -> Sum/2
  Sum/1 -> Divide/2
  Divide/1 -> Out/1

== system turbo_controller/COMMRead_ISM/ISM/AnalogFilter_T4/Subsystem1 ==
  note: 计算低通滤波中新样本的权重
      |
      | 输入T为滤波时间常数（s），T_Sampling为采样周期（s）。输出α=T_Sampling/(T+T_Sampling)，供
      | 父级乘以本拍的新输入。
      |
      | 当前T=0.067、采样周期0.02，α=0.02/0.087≈0.229885。也就是每拍只采用约23%的新值，另外约77%
      | 由历史结果补足。时间常数越大，新值权重越小，结果越平稳但响应越慢。
      |
      | 本模块只算一个无量纲系数，不含延迟，也不直接输出温度、压力或转速。两项时间输入必须使用同一
      | 单位。
  T : Inport
      settings: AttributesFormatString=T（温度、时间或真分支输入）
  T_Sampling : Inport  Port=2
      settings: AttributesFormatString=T_Sampling（采样周期）
  Constant : Constant  OutDataTypeStr=single
      settings: AttributesFormatString=Constant（常量）
  Constant2 : Constant  OutDataTypeStr=single
      settings: AttributesFormatString=Constant2（常量2）
  Divide : Product  Inputs=*/
      settings: AttributesFormatString=Divide（除法）
  Product : Product  RndMeth=Zero
      settings: AttributesFormatString=Product（乘法）
  Product1 : Product  RndMeth=Zero
      settings: AttributesFormatString=Product1（乘法1）
  Sum : Sum  Inputs=|++
      settings: AttributesFormatString=Sum（加法求和）
  Out : Outport
      settings: AttributesFormatString=Out（输出）
  wires:
  Constant/1 -> Product/1
  T_Sampling/1 -> Product/2, Sum/2
  Product/1 -> Divide/1
  Constant2/1 -> Product1/1
  T/1 -> Product1/2
  Product1/1 -> Sum/1
  Sum/1 -> Divide/2
  Divide/1 -> Out/1

== system turbo_controller/COMMRead_ISM/ISM/AnalogFilter_T4/Subsystem2 ==
  note: 计算低通滤波中历史结果的权重
      |
      | 输入T为时间常数，T_Sampling为采样周期，两者都用s。输出β=T/(T+T_Sampling)，供父级乘以上一
      | 次滤波结果。
      |
      | 当前T=0.067、采样周期0.02，β≈0.770115；与另一支路新样本权重α≈0.229885相加为1。这样常值
      | 输入最终会稳定在原值，不会因为反复相加而不断放大。
      |
      | 本模块只计算系数，历史结果由父级延迟块保存。若把20 ms误传成20 s，权重和滤波速度都会完全改
      | 变，因此父级先将Ts_ms除以1000。
  T : Inport
      settings: AttributesFormatString=T（温度、时间或真分支输入）
  T_Sampling : Inport  Port=2
      settings: AttributesFormatString=T_Sampling（采样周期）
  Constant : Constant  OutDataTypeStr=single
      settings: AttributesFormatString=Constant（常量）
  Constant2 : Constant  OutDataTypeStr=single
      settings: AttributesFormatString=Constant2（常量2）
  Divide : Product  Inputs=*/
      settings: AttributesFormatString=Divide（除法）
  Product : Product  RndMeth=Zero
      settings: AttributesFormatString=Product（乘法）
  Product1 : Product  RndMeth=Zero
      settings: AttributesFormatString=Product1（乘法1）
  Sum : Sum  Inputs=|++
      settings: AttributesFormatString=Sum（加法求和）
  Out : Outport
      settings: AttributesFormatString=Out（输出）
  wires:
  Constant/1 -> Product/1
  T/1 -> Product/2, Product1/2
  Product/1 -> Divide/1
  Constant2/1 -> Product1/1
  Product1/1 -> Sum/1
  T_Sampling/1 -> Sum/2
  Sum/1 -> Divide/2
  Divide/1 -> Out/1

== system turbo_controller/COMMRead_ISM/ISM/Origin_Nc_Filter/Subsystem1 ==
  note: 计算低通滤波中新样本的权重
      |
      | 输入T为滤波时间常数（s），T_Sampling为采样周期（s）。输出α=T_Sampling/(T+T_Sampling)，供
      | 父级乘以本拍的新输入。
      |
      | 当前T=0.067、采样周期0.02，α=0.02/0.087≈0.229885。也就是每拍只采用约23%的新值，另外约77%
      | 由历史结果补足。时间常数越大，新值权重越小，结果越平稳但响应越慢。
      |
      | 本模块只算一个无量纲系数，不含延迟，也不直接输出温度、压力或转速。两项时间输入必须使用同一
      | 单位。
  T : Inport
      settings: AttributesFormatString=T（温度、时间或真分支输入）
  T_Sampling : Inport  Port=2
      settings: AttributesFormatString=T_Sampling（采样周期）
  Constant : Constant  OutDataTypeStr=single
      settings: AttributesFormatString=Constant（常量）
  Constant2 : Constant  OutDataTypeStr=single
      settings: AttributesFormatString=Constant2（常量2）
  Divide : Product  Inputs=*/
      settings: AttributesFormatString=Divide（除法）
  Product : Product  RndMeth=Zero
      settings: AttributesFormatString=Product（乘法）
  Product1 : Product  RndMeth=Zero
      settings: AttributesFormatString=Product1（乘法1）
  Sum : Sum  Inputs=|++
      settings: AttributesFormatString=Sum（加法求和）
  Out : Outport
      settings: AttributesFormatString=Out（输出）
  wires:
  Constant/1 -> Product/1
  T_Sampling/1 -> Product/2, Sum/2
  Product/1 -> Divide/1
  Constant2/1 -> Product1/1
  T/1 -> Product1/2
  Product1/1 -> Sum/1
  Sum/1 -> Divide/2
  Divide/1 -> Out/1

== system turbo_controller/COMMRead_ISM/ISM/Origin_Nc_Filter/Subsystem2 ==
  note: 计算低通滤波中历史结果的权重
      |
      | 输入T为时间常数，T_Sampling为采样周期，两者都用s。输出β=T/(T+T_Sampling)，供父级乘以上一
      | 次滤波结果。
      |
      | 当前T=0.067、采样周期0.02，β≈0.770115；与另一支路新样本权重α≈0.229885相加为1。这样常值
      | 输入最终会稳定在原值，不会因为反复相加而不断放大。
      |
      | 本模块只计算系数，历史结果由父级延迟块保存。若把20 ms误传成20 s，权重和滤波速度都会完全改
      | 变，因此父级先将Ts_ms除以1000。
  T : Inport
      settings: AttributesFormatString=T（温度、时间或真分支输入）
  T_Sampling : Inport  Port=2
      settings: AttributesFormatString=T_Sampling（采样周期）
  Constant : Constant  OutDataTypeStr=single
      settings: AttributesFormatString=Constant（常量）
  Constant2 : Constant  OutDataTypeStr=single
      settings: AttributesFormatString=Constant2（常量2）
  Divide : Product  Inputs=*/
      settings: AttributesFormatString=Divide（除法）
  Product : Product  RndMeth=Zero
      settings: AttributesFormatString=Product（乘法）
  Product1 : Product  RndMeth=Zero
      settings: AttributesFormatString=Product1（乘法1）
  Sum : Sum  Inputs=|++
      settings: AttributesFormatString=Sum（加法求和）
  Out : Outport
      settings: AttributesFormatString=Out（输出）
  wires:
  Constant/1 -> Product/1
  T/1 -> Product1/2, Product/2
  Product/1 -> Divide/1
  Constant2/1 -> Product1/1
  Product1/1 -> Sum/1
  T_Sampling/1 -> Sum/2
  Sum/1 -> Divide/2
  Divide/1 -> Out/1

== system turbo_controller/BoardInput_输入换算与协议解析/In01_Host（上位机命令解析）/Receive（逐字节组帧与保持有效结果）_108/Step02_拼帧并记住未收完的数据/Collect（帧头识别与缓存推进）_66 ==
  note: 逐字节组帧：本页只做“找帧头、存字节、推进位置”
      |
      | 固定帧长为14字节，帧头是十六进制AA、55。输入为上一份候选缓存、已收字节数Position、本次Byte
      | 和本字节有效Active。输出为更新缓存、下一次使用的Position和本次收齐事件Complete。
      |
      | Position不是本批接收数组的序号：0表示还在找AA，1表示已见AA、正在等55，2～13表示头部已确认
      | 、继续收后面的内容。跨调用的记忆由外层Step02保存，本页根据输入计算一次更新。
      |
      | 按五步看：
      | 1 判断当前是否在等AA或55，以及字节是否匹配。
      | 2 决定这个字节应不应该进入候选缓存。
      | 3 算出本次写入位置Position+1，判断是否达到14。
      | 4 允许写入才更新对应一项，否则保留原缓存。
      | 5 按找头、重同步、收齐和无效字节规则，决定下一位置及Complete。
      |
      | 例：AA→AA→55时，第二个AA保留继续等55的机会，不当作第二帧头写入；头确认后，后续数据即使也
      | 是AA或55，仍按普通数据收下。无效字节不推进位置，也不发收齐事件。
      |
      | Complete仅表示候选帧刚拼满，不表示校验通过；外面的校验步骤还会检查内容。这里没有重写协议或
      | 增加等待时间，五步在同一次字节处理内完成。
  Buffer（上次收帧缓存）_27 : Inport  OutDataTypeStr=uint8
  Position（已收字节数）_28 : Inport  Port=2  OutDataTypeStr=uint16
  Byte（当前字节）_29 : Inport  Port=3  OutDataTypeStr=uint8
  Active（当前字节有效）_30 : Inport  Port=4  OutDataTypeStr=boolean
  Step01_判断收帧阶段与AA55 : Subsystem  Description=|
      | 第一步：看现在收到哪里，并识别AA、55
      | 
      | 只看Position和Byte，不修改缓存，不保存历史。输出三个判断：是否正在找第一个AA、当前字节是否AA、是否发生第二帧头不匹配。
      | 
      | Position=0：还没确认帧头，正在找AA。
      | Position=1：已经见到AA，期望下一个是55。
      | Position≥2：头部已确认，后续字节属于帧内数据。
      | 
      | AA是十六进制，十进制为170；55是十六进制，十进制为85。判断式：
      | 等待AA=(Position==0)；
      | 字节是AA=(Byte==170)；
      | 第二帧头错=(Position==1) AND (Byte!=85)。
      | 
      | 例：Position=1、Byte=AA时，字节是AA和第二帧头错都为真。这并不冲突：它表示没等到55，但可以把这个AA视作重新找头的机会。是否写入、位置如何调整由后面两步分别处理。
      | 
      | 本步骤不检查Active；本字节无效时，后面的写入和位置保持分支会阻止它改变状态。
  Step02_判断本字节能否写入 : Subsystem  Description=|
      | 第二步：决定本字节是否允许写进帧缓存
      | 
      | 收帧必须先找到头，所以不是每个字节都写。将第一步的三个判断与Active组合：
      | 
      | 允许写入=Active AND [
      |   (正在等AA AND 字节是AA)
      |   OR (不在等AA AND 第二帧头没有错)
      | ]。
      | 
      | 分别理解：
      | 还在找AA时，只写AA，其他噪声不进入缓存；
      | 已经见到AA、等待55时，只写正确的55；
      | 头部已经确认后，按顺序接收普通数据，不因数据恰好是AA/55就重新找头；
      | Active为假时，上述条件再合适也不写。
      | 
      | 例：已见AA后又来AA，本步骤不把第二个AA写进第2项；后面的重同步位置逻辑仍保留“已见AA”的状态，继续等55。
      | 
      | 输出只是一项布尔写许可，送第四步。它不产生新缓存，也不判断整帧校验。
  Step03_计算写入位置与是否满帧 : Subsystem  Description=|
      | 第三步：算本次写到第几项，并判断是否到帧尾
      | 
      | Position表示本次之前已接收多少项。本次候选写入位置=Position+1；帧长度固定为14，达到帧尾=(候选写入位置==14)。
      | 
      | 例如Position=0时，候选位置是1，AA应写到第1项；Position=1时，55应写到第2项；Position=13时，本次候选位置是14，这是最后一项。
      | 
      | 注意这里算的是“候选位置”：即使Active为假，仍可计算Position+1，但第四、第五步会保持缓存和位置。不能仅因候选位置等于14就认定收到新帧。
      | 
      | 候选位置送第四步写缓存；它及“达到帧尾”标志也送第五步，决定继续推进还是收齐后回0。本处不保存Position，也不清空缓存。
  Step04_写入字节或保持原缓存 : Subsystem  Description=|
      | 第四步：只更新应写的一项，其他内容保留
      | 
      | 输入包括旧缓存、本次Byte、候选写入位置和写许可。先将索引取min(候选位置,14)，防止索引超过14项缓存上界，再用Assignment生成“把这一项换成Byte”的候选数组。
      | 
      | 最终选择：写许可为真输出更新数组；写许可为假直接输出旧缓存。即使内部算出了候选更新，只要没有许可，它也不会成为输出。
      | 
      | 例：旧位置为5，本次允许接收，就把第6项换成本字节，其他13项保持；若本字节无效或第二帧头错，整份缓存保持。缓存里旧的尾部数据并不会每次清零，所以必须配合Complete和后续校验使用，不能只看数组里有值就当作新帧。
      | 
      | 本步骤不保存跨调用记忆。输出回外层的缓存记忆，供下一个字节/下一批数据继续使用。位置更新与收齐事件在第五步处理。
  Step05_更新收帧位置并报告收齐 : Subsystem  Description=|
      | 第五步：确定下一次收帧位置，并报告刚收齐
      | 
      | 先按收帧阶段选择下一Position：
      | 正在找AA：本字节是AA则到1，否则到0；
      | 正在等55但本字节不匹配：若又是AA则保持1，其他值回0；
      | 正常收数据：未到帧尾就采用Position+1，达到14项后回0，准备找下一帧头。
      | 最后再检查Active：为假时直接保留旧Position，上面的候选变化都不采用。
      | 
      | 收齐事件=Active AND 不在等待第一个AA AND 第二帧头没错 AND 达到14项。
      | 因此它只在有效字节刚补上最后一项时为真，不是缓存里有14项就一直为真。位置回0时，完整缓存仍保留供外层校验。
      | 
      | 例：Position=13，有效字节到来，输出Position=0且Complete=true；同样的位置但Active=false，则输出仍为13且Complete=false。AA、AA、55的序列依次得到位置1、1、2。
      | 
      | 本页不验证CRC或累加/异或校验，也不等待下一个20 ms节拍；Complete交外层决定是否接受这条候选帧。
  Buffer（更新后的帧缓存）_63 : Outport
  Position（下次接收位置）_64 : Outport  Port=2
  Complete（本字节组成完整帧）_65 : Outport  Port=3
  wires:
  Step05_更新收帧位置并报告收齐/2(输出2_本字节刚收齐) -> Complete（本字节组成完整帧）_65/1
  Step05_更新收帧位置并报告收齐/1(输出1_下一次已收字节数) -> Position（下次接收位置）_64/1
  Step04_写入字节或保持原缓存/1(输出1_更新后的候选缓存) -> Buffer（更新后的帧缓存）_63/1
  Step03_计算写入位置与是否满帧/1(输出1_候选位置达到帧长) -> Step05_更新收帧位置并报告收齐/3(输入3_候选位置达到帧长)  "候选位置达到帧长"
  Step03_计算写入位置与是否满帧/2(输出2_候选写入位置) -> Step04_写入字节或保持原缓存/3(输入3_候选写入位置), Step05_更新收帧位置并报告收齐/4(输入4_候选写入位置)  "候选写入位置"
  Buffer（上次收帧缓存）_27/1 -> Step04_写入字节或保持原缓存/2(输入2_上一份候选缓存)  "上一份候选缓存"
  Step02_判断本字节能否写入/1(输出1_本字节允许写缓存) -> Step04_写入字节或保持原缓存/1(输入1_本字节允许写缓存)  "本字节允许写缓存"
  Active（当前字节有效）_30/1 -> Step02_判断本字节能否写入/4(输入4_本项字节有效), Step05_更新收帧位置并报告收齐/2(输入2_本项字节有效)  "本项字节有效"
  Step01_判断收帧阶段与AA55/3(输出3_第二帧头不匹配) -> Step02_判断本字节能否写入/3(输入3_第二帧头不匹配), Step05_更新收帧位置并报告收齐/7(输入7_第二帧头不匹配)  "第二帧头不匹配"
  Step01_判断收帧阶段与AA55/1(输出1_当前字节等于AA) -> Step02_判断本字节能否写入/2(输入2_当前字节等于AA), Step05_更新收帧位置并报告收齐/1(输入1_当前字节等于AA)  "当前字节等于AA"
  Step01_判断收帧阶段与AA55/2(输出2_正在寻找第一个AA) -> Step02_判断本字节能否写入/1(输入1_正在寻找第一个AA), Step05_更新收帧位置并报告收齐/6(输入6_正在寻找第一个AA)  "正在寻找第一个AA"
  Position（已收字节数）_28/1 -> Step03_计算写入位置与是否满帧/1(输入1_本次之前已收字节数), Step05_更新收帧位置并报告收齐/5(输入5_本次之前已收字节数), Step01_判断收帧阶段与AA55/2(输入2_本次之前已收字节数)  "本次之前已收字节数"
  Byte（当前字节）_29/1 -> Step01_判断收帧阶段与AA55/1(输入1_本项字节), Step04_写入字节或保持原缓存/4(输入4_本项字节)  "本项字节"
